simulink model "pwm"  (Simulink 6.6)
settings: Solver=FixedStepDiscrete  StartTime=0.0  StopTime=1/50  FixedStep=1/100000  MaxStep=Ts  RelTol=1e-3
libraries: dsPICdrivers x3
settings Model: Creator=Administrator  LastModifiedBy=J.Vinothin Kavitha  BufferReuse=off  ProdHWDeviceType=16-bit Generic
settings DataIOCC: LimitDataPoints=off  SignalLoggingName=sigsout
settings OptimizationCC: BlockReduction=off  BooleanDataType=off  InlineInvariantSignals=on  OptimizeBlockIOStorage=off  BufferReuse=off  ExpressionFolding=off  LocalBlockOutputs=off  OptimizeModelRefInitCode=on  LifeSpan=1
settings DebuggingCC: CheckExecutionContextPreStartOutputMsg=on  CheckExecutionContextRuntimeOutputMsg=on
settings HardwareCC: ProdBitPerInt=16  ProdEndianess=LittleEndian  ProdWordSize=16  ProdHWDeviceType=16-bit Generic  TargetHWDeviceType=32-bit Generic
settings RTWCC: SystemTargetFile=dspic.tlc  TemplateMakefile=dspic_pic30_gcc.tmf  PostCodeGenCommand=dsPIC_Compile()  Description=Embedded Target for Microchip dsPIC (real-time)  ProcessScript=dspic_make_rtw_hook
settings CodeAppCC: IgnoreCustomStorageClasses=off
settings STFCustomTargetCC: TargetFcnLib=ansi_tfl_tmw.mat  GenFloatMathFcnCalls=ANSI_C  ModelReferenceCompliant=off  IncludeMdlTerminateFcn=off  CombineOutputUpdateFcns=on  ERTCustomFileBanners=on  SupportNonInlinedSFcns=off  SystemTargetFile=dspic.tlc
settings ERTTargetCC: TargetFcnLib=ansi_tfl_tmw.mat  GenFloatMathFcnCalls=ANSI_C  ModelReferenceCompliant=off  IncludeMdlTerminateFcn=off  SupportContinuousTime=on  ModelStepFunctionPrototypeControlCompliant=off  ExtMode=on  ExtModeMexFile=noextcomm  InlinedParameterPlacement=NonHierarchical  ERTSrcFileBannerTemplate=dsPIC_code_template.cgt  ERTHdrFileBannerTemplate=dsPIC_code_template.cgt  ERTDataSrcFileTemplate=dsPIC_code_template.cgt  ERTDataHdrFileTemplate=dsPIC_code_template.cgt  ERTCustomFileTemplate=dsPIC_main.tlc
settings CustomProperty: DataType=string  Value=C:\PROGRA~1\MATLAB\R2007a\rtw\bin\win32\gmake

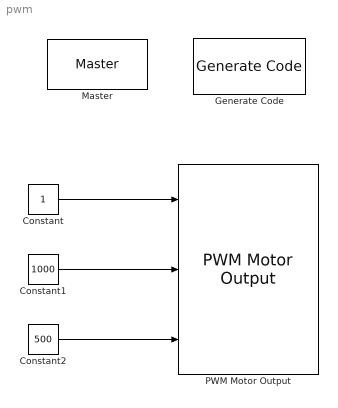
== system pwm ==
  Constant : Constant  OutDataTypeMode=boolean  SampleTime=.01
  Constant1 : Constant  Value=1000  OutDataTypeMode=uint16  SampleTime=.01
  Constant2 : Constant  Value=500  OutDataTypeMode=uint16  SampleTime=.01
  Generate Code : dsPICdrivers/Simulink Configuration/Generate Code
  Master : dsPICdrivers/Master  Tag=dsPIC_MASTER  Priority=1  TimeStepType=Free Run  picType=30f4011  fcy=10e6  Quartz_33f=5e6  PLLActive_33f=off  fcyDesired_33f=0  tmr1="[1  99  1.4211e-014]"  tmr1Info="Time Step : 1e-005  ;   Error : 1.4211e-014%  PR1=99"  tmr2345="[0  0  0  0]"  tmr2345cfg=[-1 -1 -1 -1]  IOautoConf=on  typePort="[ 0  0  0  0  0  0  0  0  0  0  0  0  0  0  0  0  0  0  0  0  0  0  0  0  0  0  0  0  0  0  0  0  0  0  0  0  0  0  0  0  0  0  0  0  0  0  0  0  0  0  0  0  0  0  0  0  0  0  0  0  0  0  0  0  0  0  0  0  0  0  0  0  0  0  0  0  0  0  0  0  0  0  0  0  0  0  0  0  0  0  0  0  0  0  0  0  0  0  0  0  0  0  0  0  0  0  0  0  0  0  0  0 ]"  TRIS="[ 65535  65535  65535  65535  65535  65535  65535 ]"  ADPCFG=0  MasterBusyPort=None  MasterOverloadPort=None  FOSC=XT_PLL8  ClockSwitchMonitor=Both disabled  TempProtection_33f=TEMP_ON  FPBOR=PBOR_OFF  PWRT=PWRT_OFF  MCLR=MCLR_EN  PowerSave=off  OverrideFcy=off  NewFcy=1e6  PR2345="[65535  65535  65535  65535]"
  PWM Motor Output : dsPICdrivers/Peripheral I//O/PWM Motor Output  Tag=dsPIC_PWM_Motor  Priority=5  PWMref=1  PWM12=1  InputEnableChk=on  InputPeriodeChk=on  Channel=[1]  TPeriode=4.194303e-001  PrescalerValue=64  PeriodeInteger=32767  MaxName='PWM'  Centered=on  HChannelON=off  Info="Nbr Bits : 16  ||  PWM = 65534  ||  Prescaler = 64"  Delay=0  IntPriority=5  nbrPwmChannelPIC=3  Status=OK  DeadTimePrescaleA=0  DeadTimePrescaleB=0  DeadTimeInfo=Dead Time A = 0  DTPWM1a=Prescaler A  DTPWM1i=Prescaler A  DTPWM2a=Prescaler A  DTPWM2i=Prescaler A  DTPWM3a=Prescaler A  DTPWM3i=Prescaler A  DTPWM4a=Prescaler A  DTPWM4i=Prescaler A  DTCON1=0  DTCON2=0
  wires:
  Constant/1 -> PWM Motor Output/1
  Constant1/1 -> PWM Motor Output/2
  Constant2/1 -> PWM Motor Output/3
